simulink model "DOF4_frequency_input"  (R2022a)
settings: Solver=FixedStepAuto  StartTime=0.0  StopTime=100  FixedStep=0.001  RelTol=1e-3
values from neighbouring files (symbols this model uses):
  a = (M_initial*a_initial + mp*xp + ml*xl) / M    (= 1.01856173677)    [DOF4_parameters.m]
  b = L - a    (= 1.62143826323)    [DOF4_parameters.m]
  cfdamper = zf*ccf    [DOF4_parameters.m]
  crdamper = zr*ccr    [DOF4_parameters.m]
  Fof = ((msf)*g)    (= 7992.92045455)    [DOF4_parameters.m]
  For = ((msr)*g)    (= 5021.02554545)    [DOF4_parameters.m]
  g = 9.81    [DOF4_parameters.m]
  I = I_initial + mp*(xp - a)^2 + ml*(xl - a)^2    (= 1798.11226226)    [DOF4_parameters.m]
  kfspring = (2*pi*ff)^2*(msf)    (= 46318.9506911)    [DOF4_parameters.m]
  krspring = ((2*pi*fr)^2)*(msr)    (= 41899.432856)    [DOF4_parameters.m]
  ktyre = 290000    [DOF4_parameters.m]
  ms = M-musf-musr    (= 1326.6)    [DOF4_parameters.m]
  musf = mu_total / 2    (= 73.7)    [DOF4_parameters.m]
  musr = mu_total / 2    (= 73.7)    [DOF4_parameters.m]
  zOftyre = (((msf)+musf)*g/ktyre)    (= 0.0300548877743)    [DOF4_parameters.m]
  zOrtyre = (((msr)+musr)*g/ktyre)    (= 0.0198069742947)    [DOF4_parameters.m]
libraries: simulink x1
settings Model: Creator=acer  LastModifiedBy=acer

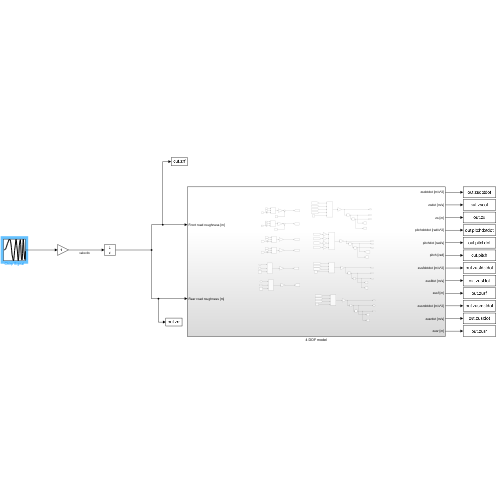
[thumbnail: Simulink's stored preview of the top-level diagram]
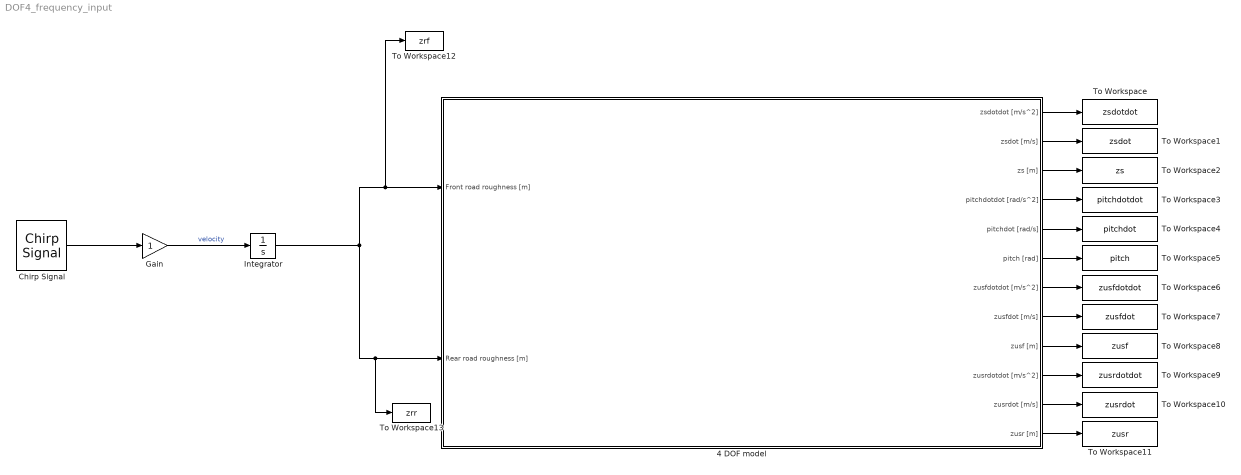
== system DOF4_frequency_input ==
  4 DOF model : Subsystem
  Chirp Signal : simulink/Sources/Chirp Signal  f1=0.1  T=100  f2=50
  Gain : Gain
  Integrator : Integrator
  To Workspace : ToWorkspace  VariableName=zsdotdot  SaveFormat=Timeseries  SampleTime=-1
  To Workspace1 : ToWorkspace  VariableName=zsdot  SaveFormat=Timeseries  SampleTime=-1
  To Workspace10 : ToWorkspace  VariableName=zusrdot  SaveFormat=Timeseries  SampleTime=-1
  To Workspace11 : ToWorkspace  VariableName=zusr  SaveFormat=Timeseries  SampleTime=-1
  To Workspace12 : ToWorkspace  VariableName=zrf  SaveFormat=Timeseries  SampleTime=-1
  To Workspace13 : ToWorkspace  VariableName=zrr  SaveFormat=Timeseries  SampleTime=-1
  To Workspace2 : ToWorkspace  VariableName=zs  SaveFormat=Timeseries  SampleTime=-1
  To Workspace3 : ToWorkspace  VariableName=pitchdotdot  SaveFormat=Timeseries  SampleTime=-1
  To Workspace4 : ToWorkspace  VariableName=pitchdot  SaveFormat=Timeseries  SampleTime=-1
  To Workspace5 : ToWorkspace  VariableName=pitch  SaveFormat=Timeseries  SampleTime=-1
  To Workspace6 : ToWorkspace  VariableName=zusfdotdot  SaveFormat=Timeseries  SampleTime=-1
  To Workspace7 : ToWorkspace  VariableName=zusfdot  SaveFormat=Timeseries  SampleTime=-1
  To Workspace8 : ToWorkspace  VariableName=zusf  SaveFormat=Timeseries  SampleTime=-1
  To Workspace9 : ToWorkspace  VariableName=zusrdotdot  SaveFormat=Timeseries  SampleTime=-1
  wires:
  4 DOF model/1(zsdotdot [m/s^2]) -> To Workspace/1
  4 DOF model/2(zsdot [m/s]) -> To Workspace1/1
  4 DOF model/3(zs [m]) -> To Workspace2/1
  4 DOF model/4(pitchdotdot [rad/s^2]) -> To Workspace3/1
  4 DOF model/5(pitchdot [rad/s]) -> To Workspace4/1
  4 DOF model/6(pitch [rad]) -> To Workspace5/1
  4 DOF model/7(zusfdotdot [m/s^2]) -> To Workspace6/1
  4 DOF model/8(zusfdot [m/s]) -> To Workspace7/1
  4 DOF model/9(zusf [m]) -> To Workspace8/1
  4 DOF model/10(zusrdotdot [m/s^2]) -> To Workspace9/1
  4 DOF model/11(zusrdot [m/s]) -> To Workspace10/1
  4 DOF model/12(zusr [m]) -> To Workspace11/1
  Chirp Signal/1 -> Gain/1
  Gain/1 -> Integrator/1  "velocity"
  Integrator/1 -> To Workspace13/1, 4 DOF model/2(Rear road roughness [m]), To Workspace12/1, 4 DOF model/1(Front road roughness [m])

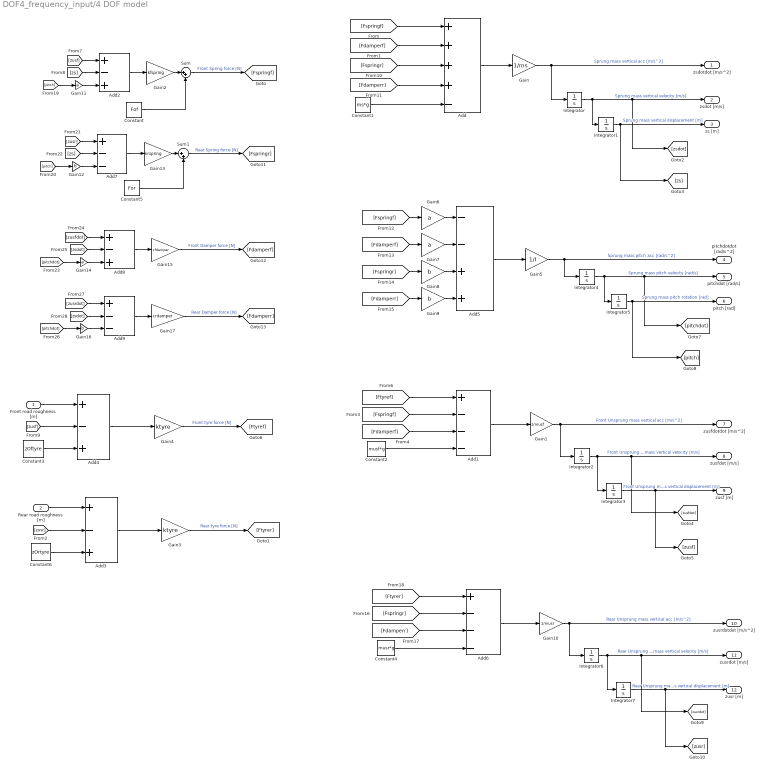
== system DOF4_frequency_input/4 DOF model ==
  Front road roughness [m] : Inport
  Rear road roughness [m] : Inport  Port=2
  Add : Sum  Inputs=++++-
  Add1 : Sum  Inputs=+---
  Add{2..4,8} (4 alike) : Sum  Inputs=+-+
  Add5 : Sum  Inputs=--++
  Add6 : Sum  Inputs=+---
  Add7 : Sum  Inputs=+--
  Add9 : Sum  Inputs=+--
  Constant : Constant  Value=Fof
  Constant1 : Constant  Value=ms*g
  Constant2 : Constant  Value=musf*g
  Constant3 : Constant  Value=zOftyre
  Constant4 : Constant  Value=musr*g
  Constant5 : Constant  Value=For
  Constant6 : Constant  Value=zOrtyre
  Gain : Gain  Gain=1/ms
  Gain1 : Gain  Gain=1/musf
  Gain10 : Gain  Gain=1/musr
  Gain{6..7,11,14} (4 alike) : Gain  Gain=a
  Gain{8..9,12,16} (4 alike) : Gain  Gain=b
  Gain13 : Gain  Gain=krspring
  Gain15 : Gain  Gain=cfdamper
  Gain17 : Gain  Gain=crdamper
  Gain2 : Gain  Gain=kfspring
  Gain3 : Gain  Gain=ktyre
  Gain4 : Gain  Gain=ktyre
  Gain5 : Gain  Gain=1/I
  Integrator{,1..7} (8 alike) : Integrator
  Sum : Sum  Inputs=|++
  Sum1 : Sum  Inputs=|++
  zsdotdot [m/s^2] : Outport
  zsdot [m/s] : Outport  Port=2
  zs [m] : Outport  Port=3
  pitchdotdot [rad/s^2] : Outport  Port=4
  pitchdot [rad/s] : Outport  Port=5
  pitch [rad] : Outport  Port=6
  zusfdotdot [m/s^2] : Outport  Port=7
  zusfdot [m/s] : Outport  Port=8
  zusf [m] : Outport  Port=9
  zusrdotdot [m/s^2] : Outport  Port=10
  zusrdot [m/s] : Outport  Port=11
  zusr [m] : Outport  Port=12
  wires:
  Sum/1 -> [Fspringf]  "Front Spring force [N]"
  [Fdamperf] -> Add1/3
  Add1/1 -> Gain1/1
  Integrator3/1 -> [zusf], zusf [m]/1  "Front Unsprung mass vertical displacement [m]"
  Gain/1 -> Integrator/1, zsdotdot [m/s^2]/1  "Sprung mass vertical acc [m/s^2]"
  Integrator2/1 -> [zusfdot], zusfdot [m/s]/1, Integrator3/1  "Front Unsprung mass vertical velocity [m/s]"
  Gain2/1 -> Sum/1
  [zs] -> Add2/2
  Constant/1 -> Sum/2
  [Fspringf] -> Add/1
  [Ftyref] -> Add1/1
  Gain1/1 -> Integrator2/1, zusfdotdot [m/s^2]/1  "Front Unsprung mass vertical acc [m/s^2]"
  [Fspringf] -> Add1/2
  Gain4/1 -> [Ftyref]  "Front tyre force [N]"
  [zusf] -> Add4/2
  Add4/1 -> Gain4/1
  Add/1 -> Gain/1
  Add2/1 -> Gain2/1
  [zusf] -> Add2/1
  [Fdamperf] -> Add/2
  Integrator1/1 -> zs [m]/1, [zs]  "Sprung mass vertical displacement [m]"
  Integrator/1 -> Integrator1/1, zsdot [m/s]/1, [zsdot]  "Sprung mass vertical velocity [m/s]"
  Constant3/1 -> Add4/3
  Constant1/1 -> Add/5
  [Fspringr] -> Add/3
  [Fdamperr] -> Add/4
  [Fdamperr] -> Gain9/1
  [Fspringr] -> Gain8/1
  Integrator4/1 -> [pitchdot], pitchdot [rad/s]/1, Integrator5/1  "Sprung mass pitch velocity [rad/s]"
  Integrator5/1 -> [pitch], pitch [rad]/1  "Sprung mass pitch rotation [rad]"
  [Fdamperf] -> Gain7/1
  Add5/1 -> Gain5/1
  [Fspringf] -> Gain6/1
  Gain5/1 -> pitchdotdot [rad/s^2]/1, Integrator4/1  "Sprung mass pitch acc [rad/s^2]"
  Gain6/1 -> Add5/1
  Gain7/1 -> Add5/2
  Gain8/1 -> Add5/3
  Gain9/1 -> Add5/4
  Constant2/1 -> Add1/4
  Constant4/1 -> Add6/4
  [Fspringr] -> Add6/2
  Gain10/1 -> zusrdotdot [m/s^2]/1, Integrator6/1  "Rear Unsprung mass vertical acc [m/s^2]"
  [Ftyrer] -> Add6/1
  Integrator6/1 -> Integrator7/1, zusrdot [m/s]/1, [zusrdot]  "Rear Unsprung mass vertical velocity [m/s]"
  Integrator7/1 -> zusr [m]/1, [zusr]  "Rear Unsprung mass vertical displacement [m]"
  Add6/1 -> Gain10/1
  [Fdamperr] -> Add6/3
  Gain11/1 -> Add2/3
  [pitch] -> Gain11/1
  [pitch] -> Gain12/1
  Gain12/1 -> Add7/3
  [zusr] -> Add7/1
  Add7/1 -> Gain13/1
  Constant5/1 -> Sum1/2
  [zs] -> Add7/2
  Gain13/1 -> Sum1/1
  Sum1/1 -> [Fspringr]  "Rear Spring force [N]"
  [pitchdot] -> Gain14/1
  Gain14/1 -> Add8/3
  [zusfdot] -> Add8/1
  Add8/1 -> Gain15/1
  [zsdot] -> Add8/2
  Gain15/1 -> [Fdamperf]  "Front Damper force [N]"
  Gain17/1 -> [Fdamperr]  "Rear Damper force [N]"
  [zsdot] -> Add9/2
  Add9/1 -> Gain17/1
  [zusrdot] -> Add9/1
  Gain16/1 -> Add9/3
  [pitchdot] -> Gain16/1
  Front road roughness [m]/1 -> Add4/1
  Rear road roughness [m]/1 -> Add3/1
  Constant6/1 -> Add3/3
  Add3/1 -> Gain3/1
  [zusr] -> Add3/2
  Gain3/1 -> [Ftyrer]  "Rear tyre force [N]"
